simulink model "MotorDC_Simulink"  (R2026a)
settings: Solver=ode45  StopTime=5
values from neighbouring files (symbols this model uses):
  b = 0.0012    [crear_motor_simscape.m]    (also in crear_motor_simulink.m; mat.m)
  J = 0.001    [crear_motor_simscape.m]    (also in crear_motor_simulink.m; mat.m)
  Ke = 0.01    [crear_motor_simscape.m]    (also in crear_motor_simulink.m; mat.m)
  Kt = 0.01    [crear_motor_simscape.m]    (also in crear_motor_simulink.m; mat.m)
  La = 0.023    [crear_motor_simscape.m]    (also in crear_motor_simulink.m; mat.m)
  Ra = 2    [crear_motor_simscape.m]    (also in crear_motor_simulink.m; mat.m)
  Tload = 0    [crear_motor_simulink.m]
  va = 12    [crear_motor_simscape.m]    (also in crear_motor_simulink.m; mat.m)
settings Model: Creator=jmlc2  LastModifiedBy=jmlc2

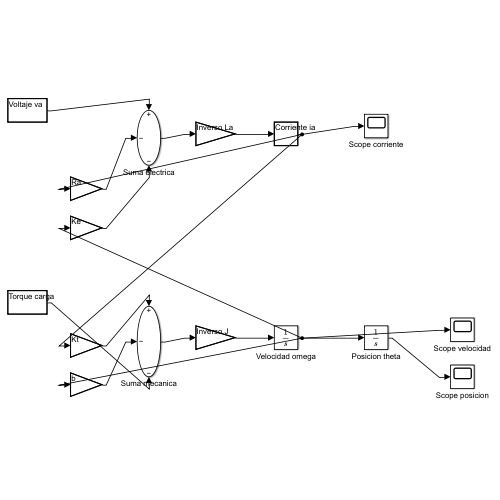
[thumbnail: Simulink's stored preview of the top-level diagram]
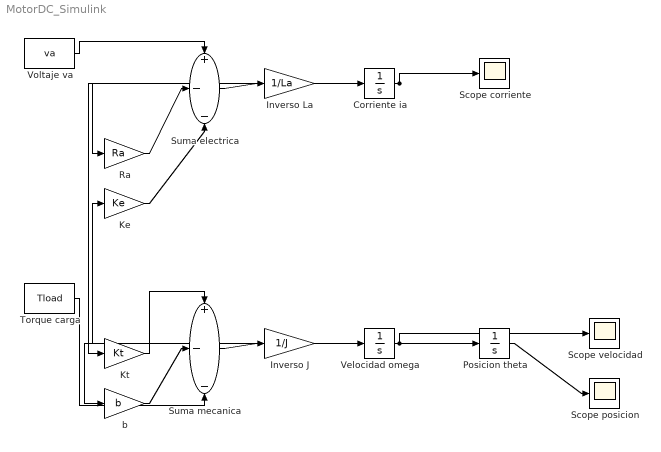
== system MotorDC_Simulink ==
  Corriente ia : Integrator
  Inverso J : Gain  Gain=1/J
  Inverso La : Gain  Gain=1/La
  Ke : Gain  Gain=Ke
  Kt : Gain  Gain=Kt
  Posicion theta : Integrator
  Ra : Gain  Gain=Ra
  Scope corriente : Scope
      settings: TimeSpan=5  ActiveDisplayYMinimum=0  ActiveDisplayYMaximum=6
  Scope posicion : Scope
      settings: TimeSpan=5  ActiveDisplayYMinimum=0  ActiveDisplayYMaximum=250
  Scope velocidad : Scope
      settings: TimeSpan=5  ActiveDisplayYMinimum=0  ActiveDisplayYMaximum=50
  Suma electrica : Sum  Inputs=+--
  Suma mecanica : Sum  Inputs=+--
  Torque carga : Constant  Value=Tload
  Velocidad omega : Integrator
  Voltaje va : Constant  Value=va
  b : Gain  Gain=b
  wires:
  Voltaje va/1 -> Suma electrica/1
  Corriente ia/1 -> Ra/1, Scope corriente/1, Kt/1
  Ra/1 -> Suma electrica/2
  Velocidad omega/1 -> Ke/1, b/1, Posicion theta/1, Scope velocidad/1
  Ke/1 -> Suma electrica/3
  Suma electrica/1 -> Inverso La/1
  Inverso La/1 -> Corriente ia/1
  Kt/1 -> Suma mecanica/1
  b/1 -> Suma mecanica/2
  Torque carga/1 -> Suma mecanica/3
  Suma mecanica/1 -> Inverso J/1
  Inverso J/1 -> Velocidad omega/1
  Posicion theta/1 -> Scope posicion/1
